simulink model "sschdlexDualActiveBridgeModel"  (R2026a)
settings: Solver=FixedStepDiscrete  StopTime=0.1  MaxStep=1/100000
PreLoadFcn:
  | Ts_FPGA = 5e-8; % FPGA Sample Time
  | Vdc = 800; % Input DC Voltage
  | L = 36e-6; % Inductance
  | N = 0.625; % Winding Ratio of the Transformer
  | Cin = 220e-6; % Input Capacitance
  | C = 470e-6; % Output Capacitance
  | R_Load = 26; % Load Resistance
  | 
  | fsw = 100000; % Switching frequency
  | period = 1/fsw; % Time period
PostLoadFcn:
  | Gs_8 = Simulink.Parameter(1e-05);
  | s_2 = Simulink.Parameter(1);
  | Gs_9 = Simulink.Parameter(0.054896);
  | Gs_10 = Simulink.Parameter(0.1758);
undefined symbols (not defined in the file or in its folder): DiscIntNeverNeededParam
libraries: SimscapeFPGAHIL_lib x16, fl_lib x13, nesl_utility x7, slpidlib x1, simulink x1, eeGeneralControl x1
settings Model: DataTypeOverride=Off  Creator=The MathWorks, Inc.  LastModifiedBy=The MathWorks, Inc.
settings SolverCC: ExtrapolationOrder=1.0  ODENIntegrationMethod=ode14x
settings OptimizationCC: ConditionallyExecuteInputs=off  InheritOutputTypeSmallerThanSingle=on
settings DebuggingCC: ArtificialAlgebraicLoopMsg=error  SingleTaskRateTransMsg=error
settings HardwareCC: ProdHWDeviceType=ASIC/FPGA->ASIC/FPGA  TargetBitPerLong=64.0  TargetBitPerPointer=64.0  TargetBitPerSizeT=64.0  TargetBitPerPtrDiffT=64.0  TargetLongLongMode=on  TargetIntDivRoundTo=Zero  TargetEndianess=LittleEndian  TargetWordSize=64.0  TargetHWDeviceType=Custom Processor->MATLAB Host Computer  ProdEqTarget=off
settings SimscapeCC: SimscapeNominalValues="[{\"value\":\"1\",\"unit\":\"A\"},{\"value\":\"1\",\"unit\":\"bar\"},{\"value\":\"1\",\"unit\":\"cm^2\"},{\"value\":\"1\",\"unit\":\"cm^3/s\"},{\"value\":\"1\",\"unit\":\"kJ/kg\"},{\"value\":\"1\",\"unit\":\"kW\"},{\"value\":\"1\",\"unit\":\"l\"},{\"value\":\"1\",\"unit\":\"N\"},{\"value\":\"1\",\"unit\":\"N*m\"},{\"value\":\"1\",\"unit\":\"V\"}]"  SimscapeLogType=none  SimscapeLogDataHistory=5000.0

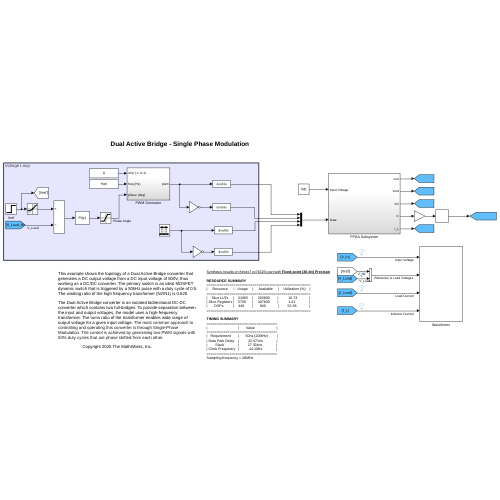
[thumbnail: Simulink's stored preview of the top-level diagram]
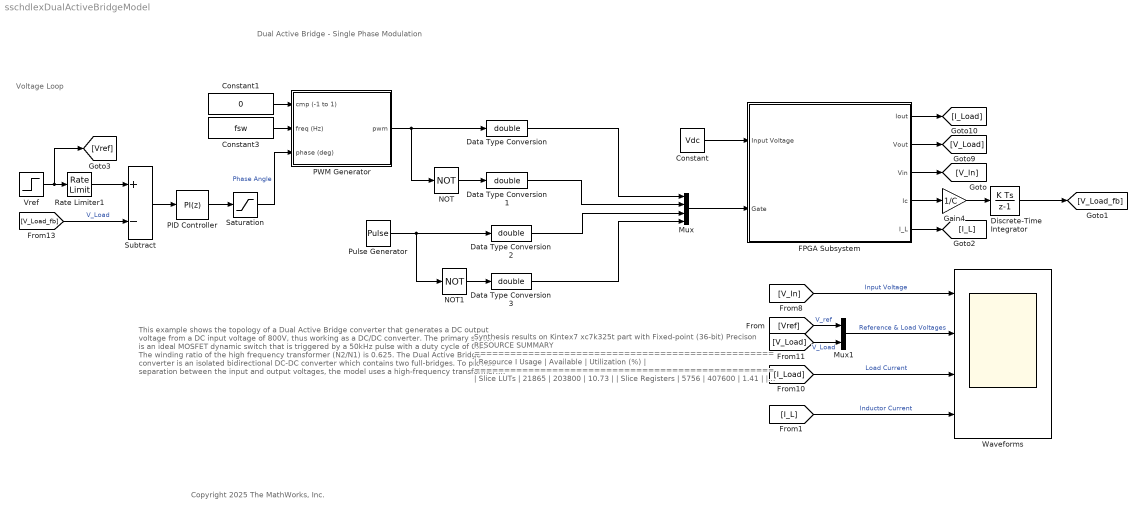
== system sschdlexDualActiveBridgeModel ==
  note: Copyright 2025 The MathWorks, Inc.
  note: Voltage Loop
  note: This example shows the topology of a Dual Active Bridge converter that generates a DC output voltage from a DC input voltage of 800V, thus working as a DC/DC converter. The primary switch is an ideal MOSFET dynamic switch that is triggered by a 50kHz pulse with a duty cycle of 0.5. The winding ratio of the high frequency transformer (N2/N1) is 0.625.
      |
      | The Dual Active Bridge converter is an isolated bidirectional DC-DC converter which contains two full-bridges. To provide separation between the input and output voltages, the model uses a high-frequency transformer. The turns ratio of the transformer enables wide range of output voltage for a given input voltage. The most common approach to controlling and operating this converter is through Single-Phase Modulation. The control is achieved by generating two PWM signals with 50% duty cycles that are phase shifted from each other.
  note: Dual Active Bridge - Single Phase Modulation
  note: Synthesis results on Kintex7 xc7k325t part with Fixed-point (36-bit) Precison
      |
      | RESOURCE SUMMARY
      | ==================================================
      | | Resource I Usage | Available | Utilization (%) |
      | ==================================================
      | | Slice LUTs | 21865 | 203800 | 10.73 |
      | | Slice Registers | 5756 | 407600 | 1.41 |
      | | DSPs | 440 | 840 | 52.38 |
      | ==================================================
      |
      | TIMING SUMMARY
      | ==================================
      | | | Value |
      | ==================================
      | | Requirement | 50ns (20MHz) |
      | | Data Path Delay | 22.471ns |
      | | Slack | 27.324ns |
      | | Clock Frequency | 44.10Hz |
      | ==================================
      | Sampling frequency = 20MHz
  Constant : Constant  Value=Vdc  SampleTime=-1
  Constant1 : Constant  Value=0  SampleTime=-1
  Constant3 : Constant  Value=fsw  SampleTime=-1
  Data Type Conversion{,1..3} (4 alike) : DataTypeConversion  OutDataTypeStr=double  SaturateOnIntegerOverflow=off  RndMeth=Floor
  Discrete-Time Integrator : DiscreteIntegrator  InitialCondition=400  SampleTime=-1  ICPrevOutput=DiscIntNeverNeededParam  ICPrevScaledInput=DiscIntNeverNeededParam
  FPGA Subsystem : Subsystem
  Gain4 : Gain  Gain=1/C
  Mux : Mux
  Mux1 : Mux  Inputs=2
  NOT : Logic  Operator=NOT  IconShape=distinctive  AllPortsSameDT=off  OutDataTypeStr=boolean
  NOT1 : Logic  Operator=NOT  IconShape=distinctive  AllPortsSameDT=off  OutDataTypeStr=boolean
  PID Controller : slpidlib/PID Controller  Controller=PI  Form=Parallel  TimeDomain=Discrete-time  UseExternalTs=off  SampleTime=-1  IntegratorMethod=Forward Euler  FilterMethod=Forward Euler  ControllerParametersSource=internal  P=0.15  I=15  UseKiTs=off  D=0  UseExternalDerivativeSource=off  N=100  UseFilter=on  TunerSelectOption=Transfer Function Based (PID Tuner App)  InitialConditionSource=internal  InitialConditionForIntegrator=0  InitialConditionForFilter=0  DifferentiatorICPrevScaledInput=0  ExternalReset=none  TrackingMode=off  Kt=1  LimitOutput=off  SatLimitsSource=internal  UpperSaturationLimit=inf  LowerSaturationLimit=-inf  LinearizeAsGain=on  AntiWindupMode=none  Kb=1  LimitIntegrator=off  UpperIntegratorSaturationLimit=inf  LowerIntegratorSaturationLimit=-inf  POutMin=[]  POutMax=[]  IOutMin=[]  IOutMax=[]  DOutMin=[]  DOutMax=[]  NOutMin=[]  NOutMax=[]  SumOutMin=[]  SumOutMax=[]  SaturationOutMin=[]  SaturationOutMax=[]  PParamMin=[]  PParamMax=[]  IParamMin=[]  IParamMax=[]  DParamMin=[]  DParamMax=[]  NParamMin=[]  NParamMax=[]  KbParamMin=[]  KbParamMax=[]  KtParamMin=[]  KtParamMax=[]  KbOutMin=[]  KbOutMax=[]  KtOutMin=[]  KtOutMax=[]  IntegratorOutMin=[]  IntegratorOutMax=[]  FilterOutMin=[]  FilterOutMax=[]  SumI1OutMin=[]  SumI1OutMax=[]  SumI2OutMin=[]  SumI2OutMax=[]  SumI3OutMin=[]  SumI3OutMax=[]  SumI4OutMin=[]  SumI4OutMax=[]  SumDOutMin=[]  SumDOutMax=[]  DifferentiatorOutMin=[]  DifferentiatorOutMax=[]  FilterDiffOutCoefMin=[]  FilterDiffOutCoefMax=[]  ReciprocalOutMin=[]  ReciprocalOutMax=[]  SumDenOutMin=[]  SumDenOutMax=[]  SumNumOutMin=[]  SumNumOutMax=[]  DivideOutMin=[]  DivideOutMax=[]  UdiffTsProdOutMin=[]  UdiffTsProdOutMax=[]  NTsProdOutMin=[]  NTsProdOutMax=[]  UintegralTsProdOutMin=[]  UintegralTsProdOutMax=[]  UngainTsProdOutMin=[]  UngainTsProdOutMax=[]  ClampingZeroOutDataTypeStr=Inherit: Inherit via back propagation  ClampingZeroOutMin=[]  ClampingZeroOutMax=[]  FilterDenConstantOutDataTypeStr=Inherit: Inherit via back propagation  FilterDenConstantOutMin=[]  FilterDenConstantOutMax=[]  PCopyOutDataTypeStr=Inherit: Inherit via back propagation  PCopyOutMin=[]  PCopyOutMax=[]  NCopyOutDataTypeStr=Inherit: Inherit via back propagation  NCopyOutMin=[]  NCopyOutMax=[]  IntegratorContinuousStateAttributes=''  IntegratorStateMustResolveToSignalObject=off  IntegratorRTWStateStorageClass=Auto  FilterContinuousStateAttributes=''  FilterStateMustResolveToSignalObject=off  FilterRTWStateStorageClass=Auto  ParallelPVariant=InternalParameters  IdealPVariant=Disabled  IVariant=InternalParameters  DVariant=Disabled  IntegratorVariant=Discrete  SatVariant=Disabled  AWVariant=Passthrough  PCopyVariant=Disabled  TRVariant=Disabled  FdbkBlocksVariant=Forward  IdealPFdbkVariant=Disabled  SatFdbkVariant=Disabled  DerivativeFilterVariant=Disabled  NVariant=Disabled  NCopyVariant=Disabled_SignalSpec  FilterICVariant=Disabled  IntegratorICVariant=InternalICs  ExternalResetVariant=Disabled  TRSumVariant=Passthrough  SumFdbkVariant=Disabled  SumVariant=Sum_PI  TsampFilterVariant=InternalTs  TsampNgainVariant=Passthrough  TsampIntegralVariant=Disabled_SignalSpec  ExternalSaturationOutDataTypeStr=Inherit: Same as second input  DerivativeSourceVariant=Disabled  PreIntVariant=InternalPreInt
  PWM Generator : Subsystem
  Pulse Generator : DiscretePulseGenerator  Period=400  PulseWidth=200  SampleTime=Ts_FPGA
  Rate Limiter1 : RateLimiter  RisingSlewLimit=fsw*2  FallingSlewLimit=-fsw*2  SampleTimeMode=inherited  InitialCondition=400
  Saturation : Saturate  UpperLimit=180  LowerLimit=0
  Subtract : Sum  Inputs=+-
  Vref : Step  Time=1/100000*10000/2  InitialValue=400  FinalValue=500  SampleTime=Ts_FPGA
  Waveforms : Scope  NumInputPorts=4
      settings: ActiveDisplayYMinimum=700  ActiveDisplayYMaximum=900
  wires:
  Constant3/1 -> PWM Generator/2(freq (Hz))
  Constant1/1 -> PWM Generator/1(cmp (-1 to 1))
  PWM Generator/1(pwm) -> Data Type Conversion/1, NOT/1
  Pulse Generator/1 -> Data Type Conversion2/1, NOT1/1
  NOT/1 -> Data Type Conversion1/1
  NOT1/1 -> Data Type Conversion3/1
  [V_In] -> Waveforms/1  "Input Voltage"
  Vref/1 -> [Vref], Rate Limiter1/1
  Subtract/1 -> PID Controller/1
  [V_Load_fb] -> Subtract/2  "V_Load"
  PID Controller/1 -> Saturation/1
  Rate Limiter1/1 -> Subtract/1
  Data Type Conversion/1 -> Mux/1
  Data Type Conversion1/1 -> Mux/2
  Data Type Conversion2/1 -> Mux/3
  Data Type Conversion3/1 -> Mux/4
  Constant/1 -> FPGA Subsystem/1(Input Voltage)
  FPGA Subsystem/1(Iout) -> [I_Load]
  FPGA Subsystem/2(Vout) -> [V_Load]
  Mux/1 -> FPGA Subsystem/2(Gate)
  FPGA Subsystem/4(Ic) -> Gain4/1
  FPGA Subsystem/3(Vin) -> [V_In]
  FPGA Subsystem/5(I_L) -> [I_L]
  [I_Load] -> Waveforms/3  "Load Current"
  Saturation/1 -> PWM Generator/3(phase (deg))  "Phase Angle"
  Gain4/1 -> Discrete-Time Integrator/1
  Discrete-Time Integrator/1 -> [V_Load_fb]
  [Vref] -> Mux1/1  "V_ref"
  [V_Load] -> Mux1/2  "V_Load"
  Mux1/1 -> Waveforms/2  "Reference & Load Voltages"
  [I_L] -> Waveforms/4  "Inductor Current"

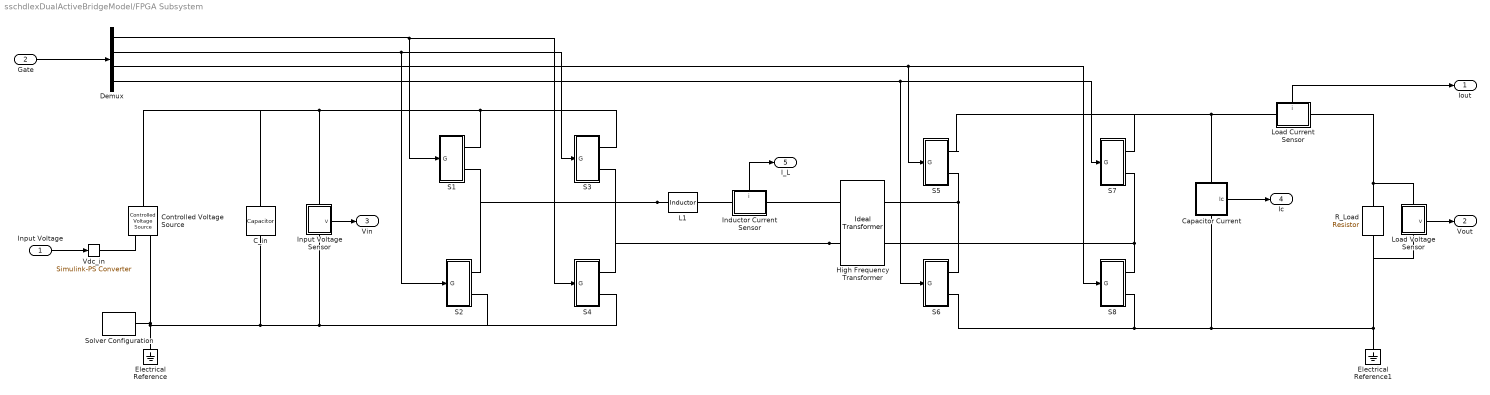
== system sschdlexDualActiveBridgeModel/FPGA Subsystem ==
  Input Voltage : Inport
  Gate : Inport  Port=2
  C_in : fl_lib/Electrical/Electrical Elements/Capacitor  c=Cin F  r=1e-6 Ohm  g=0 1/Ohm  i_specify=off  i_priority=None  i=0 A  i_nominal_specify=off  i_nominal_value=1  i_nominal_unit=A  v_specify=off  v_priority=None  v=0 V  v_nominal_specify=off  v_nominal_value=1  v_nominal_unit=V  vc_specify=on  vc_priority=High  vc=Vdc V  vc_nominal_specify=off  vc_nominal_value=1  vc_nominal_unit=V
  Capacitor Current : Subsystem
      settings: PortSchema="{\"entries\":[{\"content\":{\"sides\":[{\"content\":{\"connectorIds\":[]},\"type\":\"ConnectorPlacement.EquallySpacedRectSide\",\"uuid\":\"5da35822-cc2b-4e57-8881-bcae1460177c\"},{\"content\":{\"connectorIds\":[\"Out1\"],\"side\":\"RIGHT\"},\"type\":\"ConnectorPlacement.EquallySpacedRectSide\",\"uuid\":\"59b12fbe-0c29-41c5-8e85-a266901cfbba\"},{\"content\":{\"connectorIds\":[\"LConn1\"],\"side\":\"TOP\"},\"type\":\"ConnectorPlacement.EquallySpacedRectSide\",\"uuid\":\"d9a7ff2d-86a5-485a-93ca-f40a6f882ed3\"},{\"content\":{\"connectorIds\":[\"RConn1\"],\"side\":\"BOTTOM\"},\"type\":\"ConnectorPlacement.EquallySpacedRectSide\",\"uuid\":\"a240c809-df22-4a0d-b40f-ccc730f7bcc5\"}]},\"type\":\"ConnectorPlacement.EquallySpacedConnector\",\"uuid\":\"5bd845f1-20d5-455a-876c-e2f42d70e246\"}],\"packageUris\":[\"http://schema.mathworks.com/mf0/Connector/R2020b\"],\"version\":\"1.0\"}"
  Controlled Voltage Source : fl_lib/Electrical/Electrical Sources/Controlled Voltage Source
  Demux : Demux
  Electrical Reference : fl_lib/Electrical/Electrical Elements/Electrical Reference
  Electrical Reference1 : fl_lib/Electrical/Electrical Elements/Electrical Reference
  High Frequency Transformer : fl_lib/Electrical/Electrical Elements/Ideal Transformer  n=1/N  i1_specify=off  i1_priority=None  i1=0 A  i1_nominal_specify=off  i1_nominal_value=1  i1_nominal_unit=A  v1_specify=off  v1_priority=None  v1=0 V  v1_nominal_specify=off  v1_nominal_value=1  v1_nominal_unit=V  i2_specify=off  i2_priority=None  i2=0 A  i2_nominal_specify=off  i2_nominal_value=1  i2_nominal_unit=A  v2_specify=off  v2_priority=None  v2=0 V  v2_nominal_specify=off  v2_nominal_value=1  v2_nominal_unit=V
  Inductor Current Sensor : Subsystem
      settings: PortSchema="{\"entries\":[{\"content\":{\"sides\":[{\"content\":{\"connectorIds\":[\"LConn1\"]},\"type\":\"ConnectorPlacement.EquallySpacedRectSide\",\"uuid\":\"e9388151-e471-4783-81c5-5134e1313d7c\"},{\"content\":{\"connectorIds\":[\"RConn1\"],\"side\":\"RIGHT\"},\"type\":\"ConnectorPlacement.EquallySpacedRectSide\",\"uuid\":\"bcb23f28-0826-4736-ab91-150a314eb643\"},{\"content\":{\"connectorIds\":[\"Out1\"],\"side\":\"TOP\"},\"type\":\"ConnectorPlacement.EquallySpacedRectSide\",\"uuid\":\"e1937689-3337-4922-a316-f56c73fb0974\"}]},\"type\":\"ConnectorPlacement.EquallySpacedConnector\",\"uuid\":\"dc34a384-5aa5-46fc-88a5-47651899efae\"}],\"packageUris\":[\"http://schema.mathworks.com/mf0/Connector/R2020b\"],\"version\":\"1.0\"}"
  Input Voltage Sensor : Subsystem
      settings: PortSchema="{\"entries\":[{\"content\":{\"sides\":[{\"content\":{\"connectorIds\":[\"LConn1\"]},\"type\":\"ConnectorPlacement.EquallySpacedRectSide\",\"uuid\":\"e9388151-e471-4783-81c5-5134e1313d7c\"},{\"content\":{\"connectorIds\":[\"RConn1\"],\"side\":\"RIGHT\"},\"type\":\"ConnectorPlacement.EquallySpacedRectSide\",\"uuid\":\"bcb23f28-0826-4736-ab91-150a314eb643\"},{\"content\":{\"connectorIds\":[\"Out1\"],\"side\":\"TOP\"},\"type\":\"ConnectorPlacement.EquallySpacedRectSide\",\"uuid\":\"e1937689-3337-4922-a316-f56c73fb0974\"}]},\"type\":\"ConnectorPlacement.EquallySpacedConnector\",\"uuid\":\"dc34a384-5aa5-46fc-88a5-47651899efae\"}],\"packageUris\":[\"http://schema.mathworks.com/mf0/Connector/R2020b\"],\"version\":\"1.0\"}"
  L1 : fl_lib/Electrical/Electrical Elements/Inductor  l=L H  r=0 Ohm  g=1e-9 1/Ohm  i_specify=off  i_priority=None  i=0 A  i_nominal_specify=off  i_nominal_value=1  i_nominal_unit=A  v_specify=off  v_priority=None  v=0 V  v_nominal_specify=off  v_nominal_value=1  v_nominal_unit=V  i_L_specify=on  i_L_priority=High  i_L=0 A  i_L_nominal_specify=off  i_L_nominal_value=1  i_L_nominal_unit=A
  Load Current Sensor : Subsystem
      settings: PortSchema="{\"entries\":[{\"content\":{\"sides\":[{\"content\":{\"connectorIds\":[\"LConn1\"]},\"type\":\"ConnectorPlacement.EquallySpacedRectSide\",\"uuid\":\"e9388151-e471-4783-81c5-5134e1313d7c\"},{\"content\":{\"connectorIds\":[\"RConn1\"],\"side\":\"RIGHT\"},\"type\":\"ConnectorPlacement.EquallySpacedRectSide\",\"uuid\":\"bcb23f28-0826-4736-ab91-150a314eb643\"},{\"content\":{\"connectorIds\":[\"Out1\"],\"side\":\"TOP\"},\"type\":\"ConnectorPlacement.EquallySpacedRectSide\",\"uuid\":\"e1937689-3337-4922-a316-f56c73fb0974\"}]},\"type\":\"ConnectorPlacement.EquallySpacedConnector\",\"uuid\":\"dc34a384-5aa5-46fc-88a5-47651899efae\"}],\"packageUris\":[\"http://schema.mathworks.com/mf0/Connector/R2020b\"],\"version\":\"1.0\"}"
  Load Voltage Sensor : Subsystem
      settings: PortSchema="{\"entries\":[{\"content\":{\"sides\":[{\"content\":{\"connectorIds\":[\"LConn1\"]},\"type\":\"ConnectorPlacement.EquallySpacedRectSide\",\"uuid\":\"e9388151-e471-4783-81c5-5134e1313d7c\"},{\"content\":{\"connectorIds\":[\"RConn1\"],\"side\":\"RIGHT\"},\"type\":\"ConnectorPlacement.EquallySpacedRectSide\",\"uuid\":\"bcb23f28-0826-4736-ab91-150a314eb643\"},{\"content\":{\"connectorIds\":[\"Out1\"],\"side\":\"TOP\"},\"type\":\"ConnectorPlacement.EquallySpacedRectSide\",\"uuid\":\"e1937689-3337-4922-a316-f56c73fb0974\"}]},\"type\":\"ConnectorPlacement.EquallySpacedConnector\",\"uuid\":\"dc34a384-5aa5-46fc-88a5-47651899efae\"}],\"packageUris\":[\"http://schema.mathworks.com/mf0/Connector/R2020b\"],\"version\":\"1.0\"}"
  R_Load : fl_lib/Electrical/Electrical Elements/Resistor  R=R_Load Ohm  i_specify=off  i_priority=None  i=0 A  i_nominal_specify=off  i_nominal_value=1  i_nominal_unit=A  v_specify=off  v_priority=None  v=0 V  v_nominal_specify=off  v_nominal_value=1  v_nominal_unit=V
  S1 : Subsystem
  S2 : Subsystem
  S3 : Subsystem
  S4 : Subsystem
  S5 : Subsystem
  S6 : Subsystem
  S7 : Subsystem
  S8 : Subsystem
  Solver Configuration : nesl_utility/Solver Configuration  PhysicalDomain=network_engine_domain  SubClassName=solver  LeftPortType=input  RightPortType=generic  Tones=[]  Harmonics=[]  SimulateNoise=off  Profile=off  UseLocalSampling=off  EnableSwitchedLinearOptims=on  FrequencyDomain=off  UseCCode=off  RelTol=0.001  AbsTol=1e-06  MinStep=1e-09  ToWorkspace=off  RevertToSquareIcSolve=off  NumHomotopyIterations=100  PhasorMode=off  PhasorModeNumHarmonics=1  ConsistencySolver=NEWTON_FTOL  CanonicalOrdering=UNORDERED  OptimizeIntermediates=UNOPTIMIZED  IndexReductionMethod=DerivativeReplacement  DoDC=off  ResidualTolerance=1e-09  ConsistencyTolSource=GLOBAL  ConsistencyAbsTol=0.001  ConsistencyRelTol=0.001  ConsistencyTolFactor=0.001  UseLocalSolver=on  LocalSolverChoice=NE_BACKWARD_EULER_ADVANCER  ResolveIndetEquations=on  FunctionEvalNumThread=1  LocalSolverSampleTime=Ts_FPGA  DoFixedCost=off  MaxNonlinIter=3  MaxModeIter=2  ComputeImpulses=off  ImpulseIterations=2  LinearAlgebra=auto  LinearAlgebraNumThread=0  EquationFormulation=NE_TIME_EF  DelaysMemoryBudget=1024  AutomaticFiltering=on  FilteringTimeConstant=0.001  PartitionStorageMethod=AS_NEEDED  PartitionMemoryBudget=1024  PartitionMethod=ROBUST  MultibodyUseLocalSolver=off  MultibodyLocalSolverChoice=ODE1  MultibodyLocalSolverSampleTime=0.001
  Vdc_in : nesl_utility/Simulink-PS Converter  PhysicalDomain=network_engine_domain  SubClassName=ps_input  LeftPortType=input  RightPortType=output  PseudoPeriodic=off  Frequencies=[]  NoiseDistribution=none  NoiseParameters=[]  Unit=1  AffineConversion=off  FilteringAndDerivatives=provide  SimscapeFilterOrder=1  InputFilterTimeConstant=0.001  UdotUserProvided=0
  Iout : Outport
  Vout : Outport  Port=2
  Vin : Outport  Port=3
  Ic : Outport  Port=4
  I_L : Outport  Port=5
  wires:
  Demux/1 -> S4/1(G), S1/1(G)
  Input Voltage Sensor/1(v) -> Vin/1
  Load Current Sensor/1(i) -> Iout/1
  Load Voltage Sensor/1(v) -> Vout/1
  Capacitor Current/1(Ic) -> Ic/1
  Demux/4 -> S6/1(G), S7/1(G)
  Inductor Current Sensor/1(i) -> I_L/1
  Demux/2 -> S2/1(G), S3/1(G)
  Demux/3 -> S8/1(G), S5/1(G)
  Input Voltage/1 -> Vdc_in/1
  Gate/1 -> Demux/1
  connections:
  Load Voltage Sensor/RConn1 -- R_Load/RConn1 -- Electrical Reference1/LConn1 -- Capacitor Current/RConn1 -- S8/RConn2 -- S6/RConn2
  S5/RConn1 -- S7/RConn1 -- Capacitor Current/LConn1 -- Load Current Sensor/LConn1
  Inductor Current Sensor/RConn1 -- High Frequency Transformer/LConn1
  Input Voltage Sensor/LConn1 -- Controlled Voltage Source/LConn1 -- C_in/LConn1 -- S1/RConn1 -- S3/RConn1
  Inductor Current Sensor/LConn1 -- L1/RConn1
  Controlled Voltage Source/RConn2 -- Electrical Reference/LConn1 -- Input Voltage Sensor/RConn1 -- S2/RConn2 -- S4/RConn2 -- C_in/RConn1 -- Solver Configuration/RConn1
  R_Load/LConn1 -- Load Current Sensor/RConn1 -- Load Voltage Sensor/LConn1
  L1/LConn1 -- S1/RConn2 -- S2/RConn1
  High Frequency Transformer/RConn1 -- S5/RConn2 -- S6/RConn1
  High Frequency Transformer/RConn2 -- S7/RConn2 -- S8/RConn1
  High Frequency Transformer/LConn2 -- S3/RConn2 -- S4/RConn1
  Vdc_in/RConn1 -- Controlled Voltage Source/RConn1

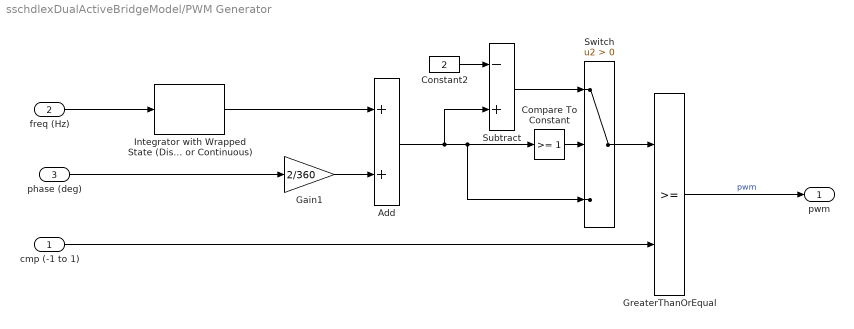
== system sschdlexDualActiveBridgeModel/PWM Generator ==
  cmp (-1 to 1) : Inport
  freq (Hz) : Inport  Port=2
  phase (deg) : Inport  Port=3
  Add : Sum
  Compare To Constant : simulink/Logic and Bit Operations/Compare To Constant  relop=>=  const=1  OutDataTypeStr=boolean
  Constant2 : Constant  Value=2  SampleTime=-1
  Gain1 : Gain  Gain=2/360
  GreaterThanOrEqual : RelationalOperator  OutDataTypeStr=boolean  RndMeth=Simplest  InputSameDT=off
  Integrator with Wrapped State (Discrete or Continuous) : eeGeneralControl/Integrator with Wrapped State (Discrete or Continuous)  LabelModeActiveChoice=Discrete  WrappedStateUpperValue=1  WrappedStateLowerValue=-1  x0=0  Ts=-1
      settings: LibrarySourceBlock=|
      | ee_sl_lib/General Control/Integrator with
      | Wrapped State
      | (Discrete or Continuous)
  Subtract : Sum  Inputs=-+
  Switch : Switch  Criteria=u2 > Threshold  SaturateOnIntegerOverflow=off  InputSameDT=off
  pwm : Outport
  wires:
  Constant2/1 -> Subtract/1
  Gain1/1 -> Add/2
  cmp (-1 to 1)/1 -> GreaterThanOrEqual/2
  Add/1 -> Switch/3, Compare To Constant/1, Subtract/2
  Compare To Constant/1 -> Switch/2
  Subtract/1 -> Switch/1
  Switch/1 -> GreaterThanOrEqual/1
  phase (deg)/1 -> Gain1/1
  GreaterThanOrEqual/1 -> pwm/1  "pwm"
  Integrator with Wrapped State (Discrete or Continuous)/1 -> Add/1
  freq (Hz)/1 -> Integrator with Wrapped State (Discrete or Continuous)/1

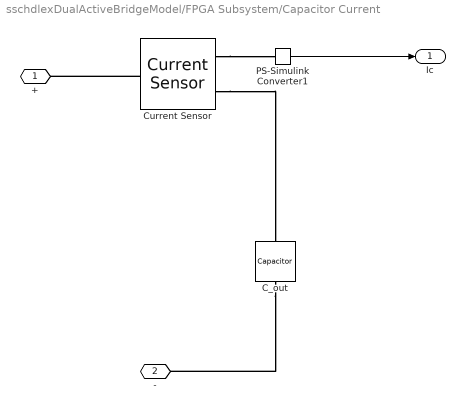
== system sschdlexDualActiveBridgeModel/FPGA Subsystem/Capacitor Current ==
  C_out : fl_lib/Electrical/Electrical Elements/Capacitor  c=C F  r=0 Ohm  g=0 1/Ohm  i_specify=off  i_priority=None  i=0 A  i_nominal_specify=off  i_nominal_value=1  i_nominal_unit=A  v_specify=off  v_priority=None  v=0 V  v_nominal_specify=off  v_nominal_value=1  v_nominal_unit=V  vc_specify=on  vc_priority=High  vc=400 V  vc_nominal_specify=off  vc_nominal_value=1  vc_nominal_unit=V
  Current Sensor : fl_lib/Electrical/Electrical Sensors/Current Sensor
  PS-Simulink Converter1 : nesl_utility/PS-Simulink Converter  PhysicalDomain=network_engine_domain  SubClassName=ps_output  LeftPortType=input  RightPortType=output  PseudoPeriodic=off  Frequencies=[]  VectorFormat=1-D array  Unit=inherit  AffineConversion=off
  + : PMIOPort  Side=Left
  - : PMIOPort  Port=2  Side=Right
  Ic : Outport
  wires:
  PS-Simulink Converter1/1 -> Ic/1
  connections:
  Current Sensor/RConn2 -- C_out/LConn1
  Current Sensor/LConn1 -- +/RConn1
  C_out/RConn1 -- -/RConn1
  Current Sensor/RConn1 -- PS-Simulink Converter1/LConn1

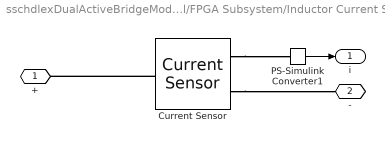
== system sschdlexDualActiveBridgeModel/FPGA Subsystem/Inductor Current Sensor ==
  Current Sensor : fl_lib/Electrical/Electrical Sensors/Current Sensor
  PS-Simulink Converter1 : nesl_utility/PS-Simulink Converter  PhysicalDomain=network_engine_domain  SubClassName=ps_output  LeftPortType=input  RightPortType=output  PseudoPeriodic=off  Frequencies=[]  VectorFormat=1-D array  Unit=inherit  AffineConversion=off
  + : PMIOPort  Side=Left
  - : PMIOPort  Port=2  Side=Right
  i : Outport
  wires:
  PS-Simulink Converter1/1 -> i/1
  connections:
  Current Sensor/RConn1 -- PS-Simulink Converter1/LConn1
  Current Sensor/LConn1 -- +/RConn1
  Current Sensor/RConn2 -- -/RConn1

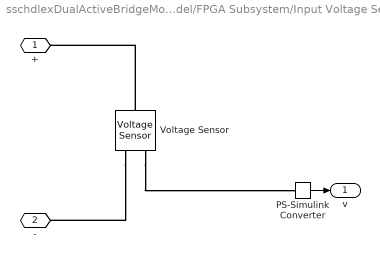
== system sschdlexDualActiveBridgeModel/FPGA Subsystem/Input Voltage Sensor ==
  PS-Simulink Converter : nesl_utility/PS-Simulink Converter  PhysicalDomain=network_engine_domain  SubClassName=ps_output  LeftPortType=input  RightPortType=output  PseudoPeriodic=off  Frequencies=[]  VectorFormat=1-D array  Unit=inherit  AffineConversion=off
  Voltage Sensor : fl_lib/Electrical/Electrical Sensors/Voltage Sensor
  + : PMIOPort  Side=Left
  - : PMIOPort  Port=2  Side=Right
  v : Outport
  wires:
  PS-Simulink Converter/1 -> v/1
  connections:
  Voltage Sensor/RConn2 -- -/RConn1
  Voltage Sensor/RConn1 -- PS-Simulink Converter/LConn1
  Voltage Sensor/LConn1 -- +/RConn1

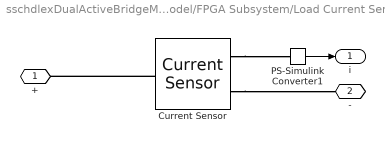
== system sschdlexDualActiveBridgeModel/FPGA Subsystem/Load Current Sensor ==
  Current Sensor : fl_lib/Electrical/Electrical Sensors/Current Sensor
  PS-Simulink Converter1 : nesl_utility/PS-Simulink Converter  PhysicalDomain=network_engine_domain  SubClassName=ps_output  LeftPortType=input  RightPortType=output  PseudoPeriodic=off  Frequencies=[]  VectorFormat=1-D array  Unit=inherit  AffineConversion=off
  + : PMIOPort  Side=Left
  - : PMIOPort  Port=2  Side=Right
  i : Outport
  wires:
  PS-Simulink Converter1/1 -> i/1
  connections:
  Current Sensor/RConn2 -- -/RConn1
  Current Sensor/LConn1 -- +/RConn1
  Current Sensor/RConn1 -- PS-Simulink Converter1/LConn1

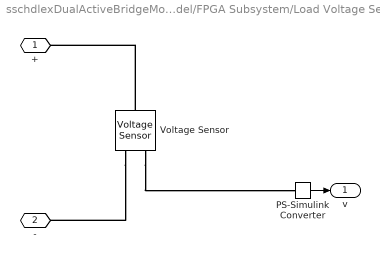
== system sschdlexDualActiveBridgeModel/FPGA Subsystem/Load Voltage Sensor ==
  PS-Simulink Converter : nesl_utility/PS-Simulink Converter  PhysicalDomain=network_engine_domain  SubClassName=ps_output  LeftPortType=input  RightPortType=output  PseudoPeriodic=off  Frequencies=[]  VectorFormat=1-D array  Unit=inherit  AffineConversion=off
  Voltage Sensor : fl_lib/Electrical/Electrical Sensors/Voltage Sensor
  + : PMIOPort  Side=Left
  - : PMIOPort  Port=2  Side=Right
  v : Outport
  wires:
  PS-Simulink Converter/1 -> v/1
  connections:
  Voltage Sensor/LConn1 -- +/RConn1
  Voltage Sensor/RConn1 -- PS-Simulink Converter/LConn1
  Voltage Sensor/RConn2 -- -/RConn1

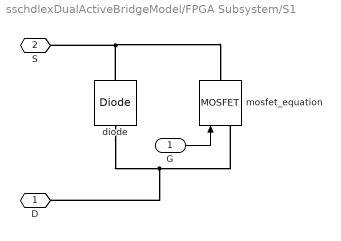
== system sschdlexDualActiveBridgeModel/FPGA Subsystem/S1 ==
  G : Inport
  diode : SimscapeFPGAHIL_lib/Dynamic Switch Models/Diode  Vf=0.8  Gs=Gs_8  s=s_2
  mosfet_equation : SimscapeFPGAHIL_lib/Dynamic Switch Models/MOSFET  Vth=0.5  Gs=Gs_9  s=s_2
  D : PMIOPort  Side=Right
  S : PMIOPort  Port=2  Side=Right
  wires:
  G/1 -> mosfet_equation/1
  connections:
  diode/LConn1 -- mosfet_equation/RConn1 -- S/RConn1
  diode/RConn1 -- mosfet_equation/LConn1 -- D/RConn1

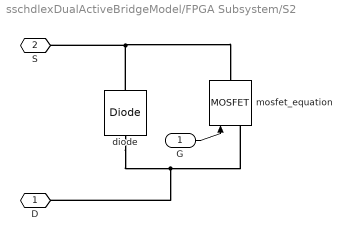
== system sschdlexDualActiveBridgeModel/FPGA Subsystem/S2 ==
  G : Inport
  diode : SimscapeFPGAHIL_lib/Dynamic Switch Models/Diode  Vf=0.8  Gs=Gs_8  s=s_2
  mosfet_equation : SimscapeFPGAHIL_lib/Dynamic Switch Models/MOSFET  Vth=0.5  Gs=Gs_9  s=s_2
  D : PMIOPort  Side=Right
  S : PMIOPort  Port=2  Side=Right
  wires:
  G/1 -> mosfet_equation/1
  connections:
  diode/LConn1 -- S/RConn1 -- mosfet_equation/RConn1
  diode/RConn1 -- mosfet_equation/LConn1 -- D/RConn1

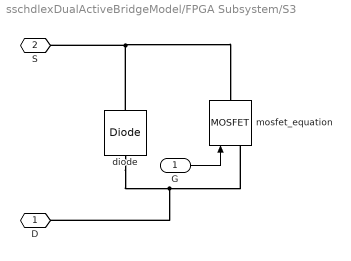
== system sschdlexDualActiveBridgeModel/FPGA Subsystem/S3 ==
  G : Inport
  diode : SimscapeFPGAHIL_lib/Dynamic Switch Models/Diode  Vf=0.8  Gs=Gs_8  s=s_2
  mosfet_equation : SimscapeFPGAHIL_lib/Dynamic Switch Models/MOSFET  Vth=0.5  Gs=Gs_9  s=s_2
  D : PMIOPort  Side=Right
  S : PMIOPort  Port=2  Side=Right
  wires:
  G/1 -> mosfet_equation/1
  connections:
  diode/RConn1 -- mosfet_equation/LConn1 -- D/RConn1
  diode/LConn1 -- mosfet_equation/RConn1 -- S/RConn1

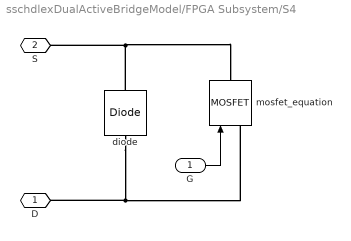
== system sschdlexDualActiveBridgeModel/FPGA Subsystem/S4 ==
  G : Inport
  diode : SimscapeFPGAHIL_lib/Dynamic Switch Models/Diode  Vf=0.8  Gs=Gs_8  s=s_2
  mosfet_equation : SimscapeFPGAHIL_lib/Dynamic Switch Models/MOSFET  Vth=0.5  Gs=Gs_9  s=s_2
  D : PMIOPort  Side=Right
  S : PMIOPort  Port=2  Side=Right
  wires:
  G/1 -> mosfet_equation/1
  connections:
  diode/RConn1 -- mosfet_equation/LConn1 -- D/RConn1
  diode/LConn1 -- S/RConn1 -- mosfet_equation/RConn1

== system sschdlexDualActiveBridgeModel/FPGA Subsystem/S5 ==
  G : Inport
  diode : SimscapeFPGAHIL_lib/Dynamic Switch Models/Diode  Vf=0.8  Gs=Gs_8  s=s_2
  mosfet_equation : SimscapeFPGAHIL_lib/Dynamic Switch Models/MOSFET  Vth=0.5  Gs=Gs_10  s=s_2
  D : PMIOPort  Side=Right
  S : PMIOPort  Port=2  Side=Right
  wires:
  G/1 -> mosfet_equation/1
  connections:
  diode/LConn1 -- mosfet_equation/RConn1 -- S/RConn1
  diode/RConn1 -- mosfet_equation/LConn1 -- D/RConn1

== system sschdlexDualActiveBridgeModel/FPGA Subsystem/S6 ==
  G : Inport
  diode : SimscapeFPGAHIL_lib/Dynamic Switch Models/Diode  Vf=0.8  Gs=Gs_8  s=s_2
  mosfet_equation : SimscapeFPGAHIL_lib/Dynamic Switch Models/MOSFET  Vth=0.5  Gs=Gs_10  s=s_2
  D : PMIOPort  Side=Right
  S : PMIOPort  Port=2  Side=Right
  wires:
  G/1 -> mosfet_equation/1
  connections:
  diode/LConn1 -- mosfet_equation/RConn1 -- S/RConn1
  diode/RConn1 -- mosfet_equation/LConn1 -- D/RConn1

== system sschdlexDualActiveBridgeModel/FPGA Subsystem/S7 ==
  G : Inport
  diode : SimscapeFPGAHIL_lib/Dynamic Switch Models/Diode  Vf=0.8  Gs=Gs_8  s=s_2
  mosfet_equation : SimscapeFPGAHIL_lib/Dynamic Switch Models/MOSFET  Vth=0.5  Gs=Gs_10  s=s_2
  D : PMIOPort  Side=Right
  S : PMIOPort  Port=2  Side=Right
  wires:
  G/1 -> mosfet_equation/1
  connections:
  diode/RConn1 -- mosfet_equation/LConn1 -- D/RConn1
  diode/LConn1 -- mosfet_equation/RConn1 -- S/RConn1

== system sschdlexDualActiveBridgeModel/FPGA Subsystem/S8 ==
  G : Inport
  diode : SimscapeFPGAHIL_lib/Dynamic Switch Models/Diode  Vf=0.8  Gs=Gs_8  s=s_2
  mosfet_equation : SimscapeFPGAHIL_lib/Dynamic Switch Models/MOSFET  Vth=0.5  Gs=Gs_10  s=s_2
  D : PMIOPort  Side=Right
  S : PMIOPort  Port=2  Side=Right
  wires:
  G/1 -> mosfet_equation/1
  connections:
  diode/RConn1 -- mosfet_equation/LConn1 -- D/RConn1
  diode/LConn1 -- mosfet_equation/RConn1 -- S/RConn1
